simulink model "THSDemo"  (R2023a)
settings: Solver=ode4  StartTime=210  StopTime=260  FixedStep=0.002  RelTol=1e-3
InitFcn:
  |  T_c = 0.002;
undefined symbols (not defined in the file or in its folder): DiscIntNeverNeededParam, Discrete, magnitude, Time
libraries: simulink x23, simulink_extras x8, sharedtransform x3, ctrlSharedLib x2, aerolibconvert2 x1, aerolibtransform2 x1, dspstat3 x1, dspsolvers x1
(part 1 of 2)
settings Model: Creator=zqinghua  LastModifiedBy=LENOVO
settings OptimizationCC: DefaultParameterBehavior=Inlined  OptimizeBlockIOStorage=off  BufferReuse=off  ReuseModelBlockBuffer=off  GlobalBufferReuse=off  ExpressionFolding=off  EnableMemcpy=off  PassReuseOutputArgsAs=Individual arguments  LocalBlockOutputs=off  ZeroExternalMemoryAtStartup=off  ZeroInternalMemoryAtStartup=off  OptimizeDataStoreBuffers=off  BusAssignmentInplaceUpdate=off  OptimizationLevel=level0  OptimizationCustomize=off  EfficientTunableParamExpr=on
settings DebuggingCC: ParameterOverflowMsg=none  ParameterUnderflowMsg=error  ParameterTunabilityLossMsg=error
settings HardwareCC: ProdBitPerInt=16  ProdBitPerPointer=16  ProdBitPerSizeT=16  ProdBitPerPtrDiffT=16  ProdLargestAtomicFloat=None  ProdWordSize=16  ProdHWDeviceType=STMicroelectronics->ST10/Super10  TargetBitPerInt=16  TargetBitPerPointer=16  TargetBitPerSizeT=16  TargetBitPerPtrDiffT=16  TargetIntDivRoundTo=Zero  TargetEndianess=LittleEndian  TargetWordSize=16  TargetHWDeviceType=STMicroelectronics->ST10/Super10
settings SFSimCC: MATLABDynamicMemAlloc=off
settings RTWCC: Description=Embedded Coder  SystemTargetFile=AFCHawk.tlc  GenCodeOnly=on  TemplateMakefile=ert_default_tmf
settings CodeAppCC: ForceParamTrailComments=on  IgnoreCustomStorageClasses=off  OperatorAnnotations=on  SimulinkDataObjDesc=on  SFDataObjDesc=on  InsertBlockDesc=on
settings STFCustomTargetCC: MultiwordLength=256  ModelReferenceCompliant=off  ConcurrentExecutionCompliant=off  CombineOutputUpdateFcns=on  ERTCustomFileBanners=on  SupportContinuousTime=off  SupportNonInlinedSFcns=off  RemoveResetFunc=on  MATLABClassNameForMDSCustomization=Simulink.SoftwareTarget.ERTCustomization  GRTInterface=off  UseToolchainInfoCompliant=off  SystemTargetFile=AFCHawk.tlc
settings ERTTargetCC: TargetLangStandard=C99 (ISO)  ModelReferenceCompliant=off  ParMdlRefBuildCompliant=off  CompOptLevelCompliant=off  ConcurrentExecutionCompliant=off  ModelStepFunctionPrototypeControlCompliant=off  CPPClassGenCompliant=off  UseToolchainInfoCompliant=off  InlinedParameterPlacement=NonHierarchical  ERTCustomFileTemplate=example_file_process.tlc

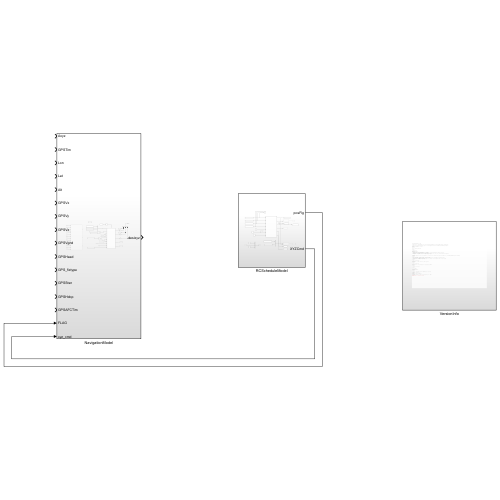
[thumbnail: Simulink's stored preview of the top-level diagram]
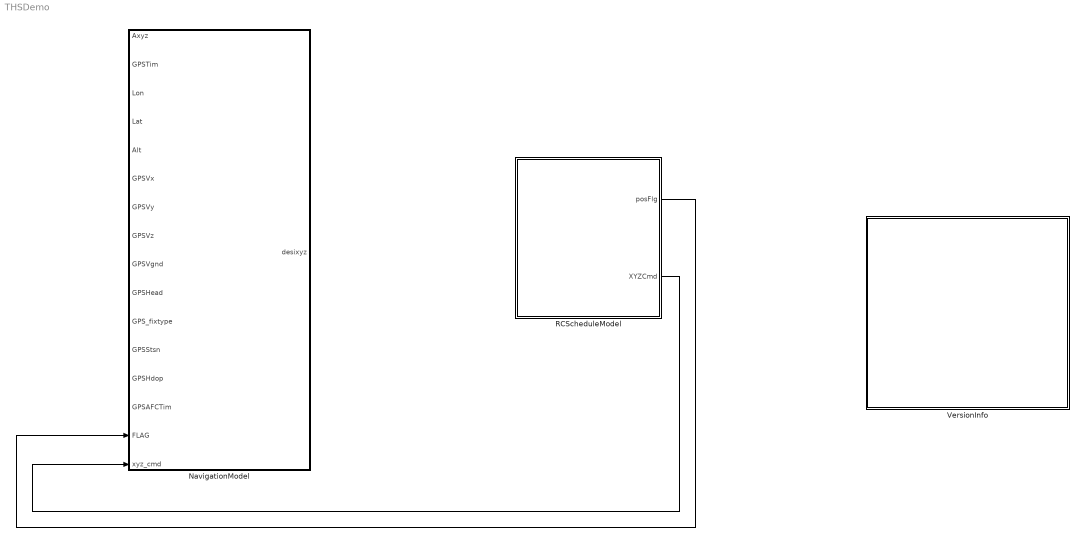
== system THSDemo ==
  NavigationModel : Subsystem
  RCScheduleModel : Subsystem
  VersionInfo : Subsystem
  wires:
  RCScheduleModel/2(XYZCmd) -> NavigationModel/16(xyz_cmd)
  RCScheduleModel/1(posFlg) -> NavigationModel/15(FLAG)

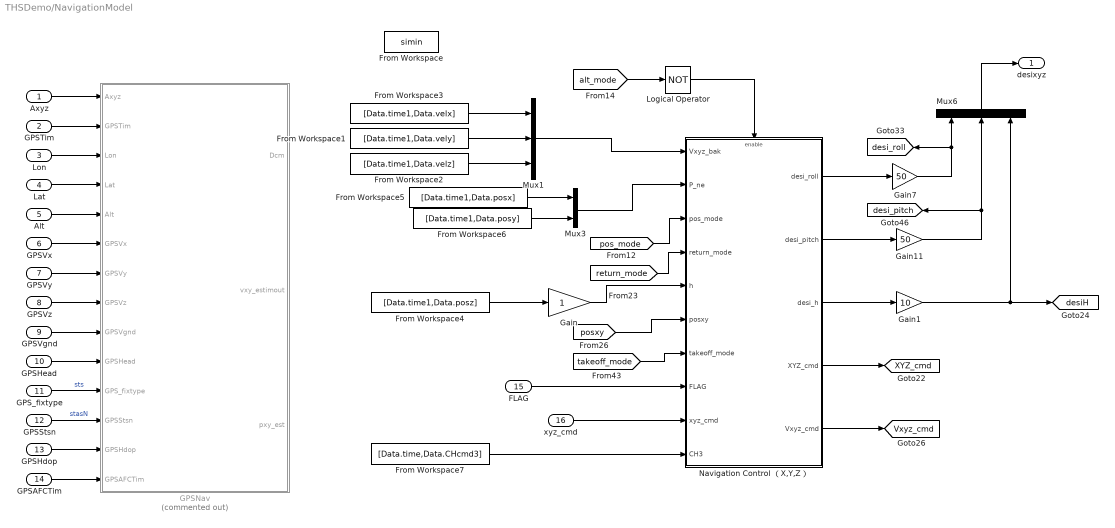
== system THSDemo/NavigationModel ==
  Axyz : Inport
  GPSTim : Inport  Port=2
  Lon : Inport  Port=3
  Lat : Inport  Port=4
  Alt : Inport  Port=5
  GPSVx : Inport  Port=6
  GPSVy : Inport  Port=7
  GPSVz : Inport  Port=8
  GPSVgnd : Inport  Port=9
  GPSHead : Inport  Port=10
  GPS_fixtype : Inport  Port=11
  GPSStsn : Inport  Port=12
  GPSHdop : Inport  Port=13
  GPSAFCTim : Inport  Port=14
  FLAG : Inport  Port=15
  xyz_cmd : Inport  Port=16
  " Navigation Control （X,Y,Z）" : Subsystem
  From Workspace : FromWorkspace  VariableName=simin
  From Workspace1 : FromWorkspace  VariableName=[Data.time1,Data.vely]
  From Workspace2 : FromWorkspace  VariableName=[Data.time1,Data.velz]
  From Workspace3 : FromWorkspace  VariableName=[Data.time1,Data.velx]
  From Workspace4 : FromWorkspace  VariableName=[Data.time1,Data.posz]
  From Workspace5 : FromWorkspace  VariableName=[Data.time1,Data.posx]
  From Workspace6 : FromWorkspace  VariableName=[Data.time1,Data.posy]
  From Workspace7 : FromWorkspace  VariableName=[Data.time,Data.CHcmd3]
  GPSNav : Subsystem  Commented=on
  Gain : Gain
  Gain1 : Gain  Gain=10
  Gain11 : Gain  Gain=50
  Gain7 : Gain  Gain=50
  Logical Operator : Logic  Operator=NOT  AllPortsSameDT=off  OutDataTypeStr=boolean
  Mux1 : Mux  Inputs=3
  Mux3 : Mux  Inputs=2
  Mux6 : Mux  Inputs=3
  desixyz : Outport
  tag scope: Vxyz_cmd=global, XYZ_cmd=global, desiH=global, desi_pitch=global, desi_roll=global
  wires:
  xyz_cmd/1 -> " Navigation Control （X,Y,Z）"/9(xyz_cmd)
  Mux6/1 -> desixyz/1
  FLAG/1 -> " Navigation Control （X,Y,Z）"/8(FLAG)
  Gain1/1 -> Mux6/3, [desiH]
  From Workspace4/1 -> Gain/1
  [takeoff_mode] -> " Navigation Control （X,Y,Z）"/7(takeoff_mode)
  " Navigation Control （X,Y,Z）"/3(desi_h) -> Gain1/1
  [pos_mode] -> " Navigation Control （X,Y,Z）"/3(pos_mode)
  Logical Operator/1 -> " Navigation Control （X,Y,Z）"/Enable
  [return_mode] -> " Navigation Control （X,Y,Z）"/4(return_mode)
  Gain/1 -> " Navigation Control （X,Y,Z）"/5(h)
  [posxy] -> " Navigation Control （X,Y,Z）"/6(posxy)
  " Navigation Control （X,Y,Z）"/1(desi_roll) -> Gain7/1
  " Navigation Control （X,Y,Z）"/2(desi_pitch) -> Gain11/1
  " Navigation Control （X,Y,Z）"/4(XYZ_cmd) -> [XYZ_cmd]
  " Navigation Control （X,Y,Z）"/5(Vxyz_cmd) -> [Vxyz_cmd]
  Gain7/1 -> Mux6/1, [desi_roll]
  Gain11/1 -> Mux6/2, [desi_pitch]
  GPSTim/1 -> GPSNav/2(GPSTim)
  Lon/1 -> GPSNav/3(Lon)
  Lat/1 -> GPSNav/4(Lat)
  Alt/1 -> GPSNav/5(Alt)
  GPSVx/1 -> GPSNav/6(GPSVx)
  GPSVy/1 -> GPSNav/7(GPSVy)
  GPSVz/1 -> GPSNav/8(GPSVz)
  GPSVgnd/1 -> GPSNav/9(GPSVgnd)
  GPSHead/1 -> GPSNav/10(GPSHead)
  GPS_fixtype/1 -> GPSNav/11(GPS_fixtype)  "sts"
  GPSStsn/1 -> GPSNav/12(GPSStsn)  "stasN"
  GPSHdop/1 -> GPSNav/13(GPSHdop)
  GPSAFCTim/1 -> GPSNav/14(GPSAFCTim)
  [alt_mode] -> Logical Operator/1
  Axyz/1 -> GPSNav/1(Axyz)
  From Workspace7/1 -> " Navigation Control （X,Y,Z）"/10(CH3)
  Mux1/1 -> " Navigation Control （X,Y,Z）"/1(Vxyz_bak)
  From Workspace3/1 -> Mux1/1
  From Workspace1/1 -> Mux1/2
  From Workspace2/1 -> Mux1/3
  Mux3/1 -> " Navigation Control （X,Y,Z）"/2(P_ne)
  From Workspace6/1 -> Mux3/2
  From Workspace5/1 -> Mux3/1

== system THSDemo/RCScheduleModel ==
  Constant{,4,7..10} (6 alike) : Constant  Value=0
  From Workspace1 : FromWorkspace  VariableName=[Data.time,Data.ch5]
  From Workspace2 : FromWorkspace  VariableName=[Data.time,Data.ch6]
  From Workspace3 : FromWorkspace  VariableName=[Data.time,Data.ch8]
  From Workspace4 : FromWorkspace  VariableName=[Data.time,Data.ch7]
  From Workspace5 : FromWorkspace  VariableName=[Data.time1,Data.posx]
  From Workspace6 : FromWorkspace  VariableName=[Data.time1,Data.posy]
  Goto27 : Goto  Commented=on  GotoTag=pos_mode_alt
  Goto28 : Goto  Commented=on  GotoTag=posz
  Mux2 : Mux  Inputs=3
  Mux3 : Mux  Inputs=2
  Scope : Scope  NumInputPorts=4
  Subsystem : Subsystem  Commented=on
  Subsystem1 : Subsystem  Commented=on
  control_mode : Subsystem
  posFlg : Outport
  XYZCmd : Outport  Port=2
  tag scope: alt_mode=global, pos_mode=global, posxy=global, return_mode=global, sbus_init_ESC=global, takeoff_mode=global
  wires:
  Mux3/1 -> Subsystem/1(pos)
  Constant/1 -> posFlg/1, control_mode/6(pos_flag)
  Constant7/1 -> Mux2/2
  Constant4/1 -> Mux2/1
  Constant8/1 -> Mux2/3
  From Workspace3/1 -> Scope/4, control_mode/1(sbus_return)
  control_mode/4(pos_mode_alt) -> Goto27/1
  control_mode/3(takeoff_mode) -> [takeoff_mode], Subsystem1/2(pos_mode_0)
  From Workspace4/1 -> Scope/3, control_mode/2(sbus_pos)
  From Workspace2/1 -> Scope/2, control_mode/3(sbus_alt)
  control_mode/1(return_mode) -> Subsystem/2(return), [return_mode]
  control_mode/2(pos_mode) -> [pos_mode]
  control_mode/5(master_alt_mode) -> [alt_mode]
  control_mode/6(sbus_init&ESC1) -> [sbus_init_ESC]
  Subsystem1/1(posz) -> Goto28/1
  Subsystem/1(posxy) -> [posxy]
  Mux2/1 -> XYZCmd/1
  Constant9/1 -> control_mode/5(return_flag)
  Constant10/1 -> control_mode/7(take_off_flag)
  From Workspace5/1 -> Mux3/1
  From Workspace6/1 -> Mux3/2
  From Workspace1/1 -> Scope/1, control_mode/4(sbus_init&ESC)

== system THSDemo/VersionInfo ==
  note: % 2024-01-11 Positon Controller 修改 ， by REZ
      |
      | 1.积分器重置条件，根据油门，已知实际遥控器CH3>0.4左右开始离地，离地前需要进行积分器重置； 遥控器的CH3=0.3-0.4左右对应在模型中Cmd_ch3=880，即重置条件为：当Ch3<880进行积分重置。
      |
      | 2.积分器的限幅范围：对位置控制器里的四个积分器暂时施加了[-3,3]的限幅，主要考虑当x和y方向的位置误差最大在3m内的时候，单纯由积分器得到的控制量不能占据PID控制器主导量而导致控制异常！
      |
      | %2024-01-15:
      | 位置控制器重修，P-PID控制器参数修改了一版；积分限幅
      |
      | % 2024-01-16：
      | 修改增加了一个含逻辑切换的正方形航迹规划指令；
      |
      | %2024-01-19:
      | 航迹规划的优化及飞行验证；
      |
      | %22024-03-08：
      | 增加control_mode模式选择模块：
      | （1）ch5为sbus_init_ESC开关同时进行电调控制解锁与导航初始化，其不受其他模式影响；
      | （2）ch6为高度控制与位置模式的切换通道，通道置1为高度控制模式，否则将进行位置控制模式，在所有模式中高度控制模式优先级最高，只要该通道置1，其他模式将不起作用；
      | （3）ch7为位置控制模式，该模式优先级最低，主要进行航迹飞行，其他通道置零，ch7通道置1，进行预设点飞行，否则进入（0,0,h）定点模式，定点模式可以理解为航迹规划前的无人机位置调整与准备；
      | （4）ch8为返航控制模式，该模式优先级高于航迹控制，但低于高度控制模式，通道置1，无人机将进行返航任务。
      |
      | %22024-03-08：
      | 优化位置控制模块，可随意更改航迹点，并预留与上位机进行点位设置的接口模块。 注意 ，该版本航迹飞行为平面飞行，未涉及到高度，因此在进行点位设置时，只需设计X和Y两个方向的点位，可自行在setpoints封装模块的MASK界面进行修改，同时可修改触发阈值。
      |
      | %22024-03-10：
      | 优化位置控制，同时增加返航模块。将位置控制模式划分为三个模 式，（0,0）定点模式，航迹规划模式，一键返航模式，与control_mode相对应，通过遥控器对应拨杆进行模式切换。
      | （1）三个模式共用同一组控制参数，（0,0）定点模式和航迹规划模式不进行高度控制，保持当前高度；
      | （2）一键返航模式任务要求，无人机接收到指令后，首先保持水平位置，进行高度方向的飞行，达到决断高度之后，无人机保持当前高度h0,然后向（0,0,h）点位飞行，随后无人机进行降落。
      | （3）将位置模式产生的上升率与下降率叠加到遥控器指令生成的控制率中。
      |
      | %22024-03-11：
      | 优化位置控制，可进行三维空间点位设置。
      |
      | %22024-03-12：
      | 取消pos_mode(0,0)模式，优化三维航迹，无人机接受指令后，先飞行高度，随后进行水平飞行。
      |
      | %22024-03-14：
      | 优化返航模式，解决了返航复飞的现象。
      |
      | %22024-03-14：
      | 增加了定点模式，航迹飞行前，无人机先进行当前高度的单定点飞行，验证其飞行性能，随后进行三维航迹飞行。
      |
      | %22024-03-14：
      | 加入偏航控制模式，使其一直处于正北方向。
      |
      | %22024-03-15：
      | 增加上位机点位设置模块。
      |
      | %22024-03-16：
      | 将偏航控制单独加到位置控制模式；
      |
      | %22024-03-17：
      | 增加一键起飞模式，无人机解锁，同时油门至中位，此时，将遥控器7号拨杆至中位，无人机进行一键起飞。
      |
      | %22024-03-18：
      | 简化三维航迹飞行，同时进行高度与水平飞行。
      | %22024-03-22：
      | 优化偏航控制，在飞行高度大于0.5米，偏航控制有效。
      | %22024-03-24：
      | 优化上位机控制逻辑，实现遥控控制与上位机控制相互兼容，上位机可发送起飞指令，返航指令，三维坐标点。
      | %22024-05-15:
      | F550-4 飞8m；未加磁力计补偿，yaw的kp参数需要在线调参为6.6；

== system THSDemo/NavigationModel/ Navigation Control （X,Y,Z） ==
  Vxyz_bak : Inport
  P_ne : Inport  Port=2
  pos_mode : Inport  Port=3
  return_mode : Inport  Port=4
  h : Inport  Port=5
  posxy : Inport  Port=6
  takeoff_mode : Inport  Port=7
  FLAG : Inport  Port=8
  xyz_cmd : Inport  Port=9
  CH3 : Inport  Port=10
  Enable : EnablePort
  POS_CONTROL : Subsystem
  POS_PID : Subsystem
  SETPOINT_z1 : Subsystem
  Scope : Scope  NumInputPorts=2
  Scope1 : Scope  NumInputPorts=2
  desi_roll : Outport
  desi_pitch : Outport  Port=2
  desi_h : Outport  Port=3
  XYZ_cmd : Outport  Port=4
  Vxyz_cmd : Outport  Port=5
  wires:
  POS_PID/1(desi_roll) -> desi_roll/1
  POS_PID/2(desi_pitch) -> desi_pitch/1
  POS_PID/3(desi_h) -> desi_h/1
  return_mode/1 -> SETPOINT_z1/3(return_mode)
  pos_mode/1 -> SETPOINT_z1/2(pos_mode)
  SETPOINT_z1/1(XYZ_cmd) -> POS_CONTROL/1(XYZ_cmd), Scope1/1, XYZ_cmd/1
  P_ne/1 -> SETPOINT_z1/4(pos), Scope1/2, POS_CONTROL/2(pos)
  h/1 -> POS_CONTROL/3(h), SETPOINT_z1/5(h)
  POS_CONTROL/1(Vxyz_cmd) -> POS_PID/1(Vxyz_cmd), Scope/1, Vxyz_cmd/1
  posxy/1 -> SETPOINT_z1/1(posxy)
  takeoff_mode/1 -> SETPOINT_z1/6(takeoff_mode)
  xyz_cmd/1 -> SETPOINT_z1/7(xyz_cmd)
  FLAG/1 -> SETPOINT_z1/8(FLAG)
  CH3/1 -> POS_PID/3(CH3)
  Vxyz_bak/1 -> Scope/2, POS_PID/2(Vxyz_bak)

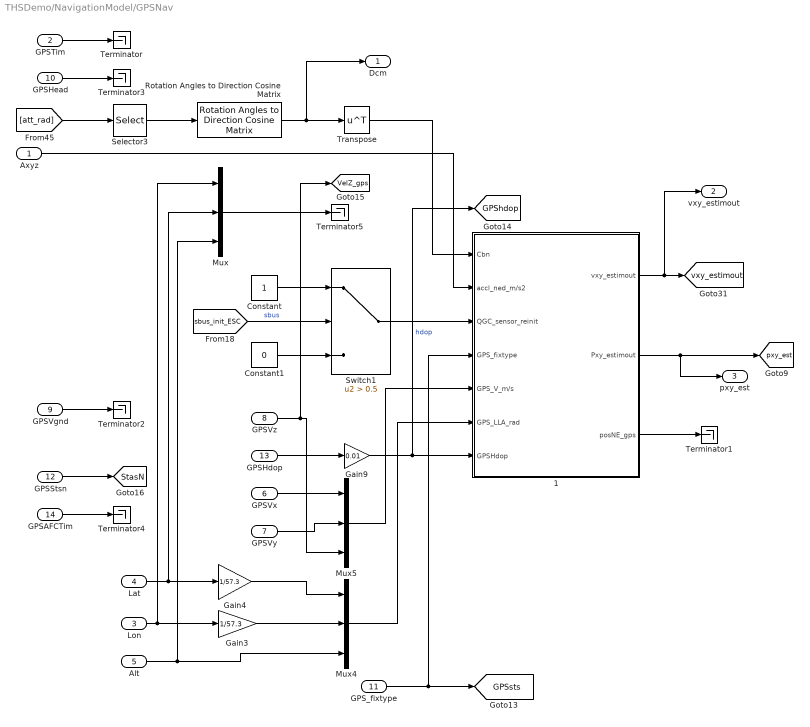
== system THSDemo/NavigationModel/GPSNav ==
  Axyz : Inport
  GPSTim : Inport  Port=2
  Lon : Inport  Port=3
  Lat : Inport  Port=4
  Alt : Inport  Port=5
  GPSVx : Inport  Port=6
  GPSVy : Inport  Port=7
  GPSVz : Inport  Port=8
  GPSVgnd : Inport  Port=9
  GPSHead : Inport  Port=10
  GPS_fixtype : Inport  Port=11
  GPSStsn : Inport  Port=12
  GPSHdop : Inport  Port=13
  GPSAFCTim : Inport  Port=14
  1 : Subsystem  mask{dt=0.002}
      mask prompts: dt "步长"
      mask DialogControl ParameterGroupVar Prompt: 参数
  Constant : Constant
  Constant1 : Constant  Value=0
  Gain3 : Gain  Gain=1/57.3
  Gain4 : Gain  Gain=1/57.3
  Gain9 : Gain  Gain=0.01
  Mux : Mux  Inputs=3
  Mux4 : Mux  Inputs=3
  Mux5 : Mux  Inputs=3
  Rotation Angles to Direction Cosine Matrix : sharedtransform/Rotation Angles to Direction Cosine Matrix  rotationOrder=ZYX  aMode=aMode
  Selector3 : Selector  InputPortWidth=3  IndexOptions=Index vector (dialog)  Indices=[3 2 1]  OutputSizes=1
  Switch1 : Switch  Criteria=u2 > Threshold  Threshold=0.5  SaturateOnIntegerOverflow=off  InputSameDT=off
  Terminator{,1..5} (6 alike) : Terminator
  Transpose : Math  Operator=transpose
  Dcm : Outport
  vxy_estimout : Outport  Port=2
  pxy_est : Outport  Port=3
  tag scope: GPShdop=global, GPSsts=global, StasN=global, VelZ_gps=global, pxy_est=global, vxy_estimout=global
  wires:
  GPSTim/1 -> Terminator/1
  GPSVz/1 -> [VelZ_gps], Mux5/3
  GPSStsn/1 -> [StasN]
  GPSVgnd/1 -> Terminator2/1
  GPSHead/1 -> Terminator3/1
  Gain3/1 -> Mux4/2
  Mux/1 -> Terminator5/1
  [att_rad] -> Selector3/1
  Selector3/1 -> Rotation Angles to Direction Cosine Matrix/1
  Axyz/1 -> 1/2(accl_ned_m/s2)
  GPSAFCTim/1 -> Terminator4/1
  Lat/1 -> Gain4/1, Mux/2
  GPSVy/1 -> Mux5/2
  Lon/1 -> Gain3/1, Mux/1
  Alt/1 -> Mux4/3, Mux/3
  Rotation Angles to Direction Cosine Matrix/1 -> Transpose/1, Dcm/1
  Constant1/1 -> Switch1/3
  [sbus_init_ESC] -> Switch1/2  "sbus"
  Constant/1 -> Switch1/1
  GPSHdop/1 -> Gain9/1
  GPSVx/1 -> Mux5/1
  Gain4/1 -> Mux4/1
  Transpose/1 -> 1/1(Cbn)
  Switch1/1 -> 1/3(QGC_sensor_reinit)
  Mux4/1 -> 1/6(GPS_LLA_rad)
  Gain9/1 -> 1/7(GPSHdop), [GPShdop]  "hdop"
  Mux5/1 -> 1/5(GPS_V_m/s)
  GPS_fixtype/1 -> [GPSsts], 1/4(GPS_fixtype)
  1/1(vxy_estimout) -> [vxy_estimout], vxy_estimout/1
  1/2(Pxy_estimout) -> pxy_est/1, [pxy_est]
  1/3(posNE_gps) -> Terminator1/1

== system THSDemo/RCScheduleModel/Subsystem ==
  pos : Inport
  return : Inport  Port=2
  Logical Operator : Logic  Operator=NOT  AllPortsSameDT=off  OutDataTypeStr=boolean
  Memory : Memory
  Switch : Switch  Criteria=u2 > Threshold  Threshold=0.5  SaturateOnIntegerOverflow=off  InputSameDT=off
  posxy : Outport
  wires:
  Switch/1 -> Memory/1, posxy/1
  Memory/1 -> Switch/3
  return/1 -> Logical Operator/1
  pos/1 -> Switch/1
  Logical Operator/1 -> Switch/2

== system THSDemo/RCScheduleModel/Subsystem1 ==
  h : Inport
  pos_mode_0 : Inport  Port=2
  Gain : Gain  Gain=-0.01
  Logical Operator : Logic  Operator=NOT  AllPortsSameDT=off  OutDataTypeStr=boolean
  Memory : Memory
  Switch : Switch  Criteria=u2 > Threshold  Threshold=0.5  SaturateOnIntegerOverflow=off  InputSameDT=off
  posz : Outport
  wires:
  Logical Operator/1 -> Switch/2
  h/1 -> Gain/1
  pos_mode_0/1 -> Logical Operator/1
  Memory/1 -> Switch/3
  Switch/1 -> posz/1, Memory/1
  Gain/1 -> Switch/1

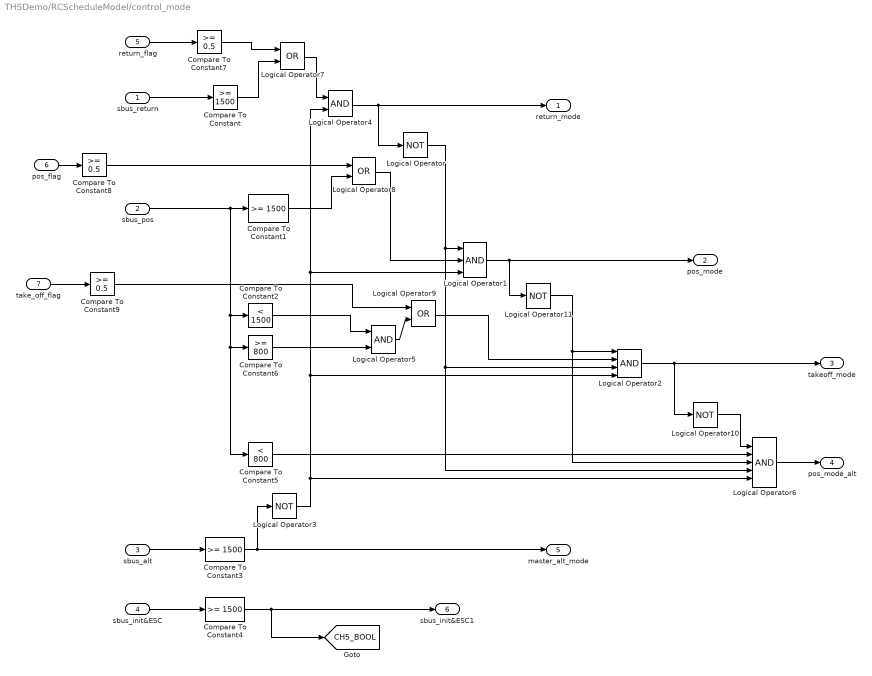
== system THSDemo/RCScheduleModel/control_mode ==
  sbus_return : Inport
  sbus_pos : Inport  Port=2
  sbus_alt : Inport  Port=3
  sbus_init&ESC : Inport  Port=4
  return_flag : Inport  Port=5
  pos_flag : Inport  Port=6
  take_off_flag : Inport  Port=7
  Compare To Constant{,1,3..4} (4 alike) : simulink/Logic and Bit Operations/Compare To Constant  relop=>=  const=1500  OutDataTypeStr=boolean
  Compare To Constant2 : simulink/Logic and Bit Operations/Compare To Constant  relop=<  const=1500  OutDataTypeStr=boolean
  Compare To Constant5 : simulink/Logic and Bit Operations/Compare To Constant  relop=<  const=800  OutDataTypeStr=boolean
  Compare To Constant6 : simulink/Logic and Bit Operations/Compare To Constant  relop=>=  const=800  OutDataTypeStr=boolean
  Compare To Constant7 : simulink/Logic and Bit Operations/Compare To Constant  relop=>=  const=0.5  OutDataTypeStr=boolean
  Compare To Constant8 : simulink/Logic and Bit Operations/Compare To Constant  relop=>=  const=0.5  OutDataTypeStr=boolean
  Compare To Constant9 : simulink/Logic and Bit Operations/Compare To Constant  relop=>=  const=0.5  OutDataTypeStr=boolean
  Logical Operator{,3,10..11} (4 alike) : Logic  Operator=NOT  AllPortsSameDT=off  OutDataTypeStr=boolean
  Logical Operator1 : Logic  Inputs=3  AllPortsSameDT=off  OutDataTypeStr=boolean
  Logical Operator2 : Logic  Inputs=4  AllPortsSameDT=off  OutDataTypeStr=boolean
  Logical Operator4 : Logic  AllPortsSameDT=off  OutDataTypeStr=boolean
  Logical Operator5 : Logic  AllPortsSameDT=off  OutDataTypeStr=boolean
  Logical Operator6 : Logic  Inputs=5  AllPortsSameDT=off  OutDataTypeStr=boolean
  Logical Operator7 : Logic  Operator=OR  AllPortsSameDT=off  OutDataTypeStr=boolean
  Logical Operator8 : Logic  Operator=OR  AllPortsSameDT=off  OutDataTypeStr=boolean
  Logical Operator9 : Logic  Operator=OR  AllPortsSameDT=off  OutDataTypeStr=boolean
  return_mode : Outport
  pos_mode : Outport  Port=2
  takeoff_mode : Outport  Port=3
  pos_mode_alt : Outport  Port=4
  master_alt_mode : Outport  Port=5
  sbus_init&ESC1 : Outport  Port=6
  tag scope: CH5_BOOL=global
  wires:
  Logical Operator4/1 -> Logical Operator/1, return_mode/1
  Logical Operator/1 -> Logical Operator6/4, Logical Operator2/3, Logical Operator1/1
  sbus_return/1 -> Compare To Constant/1
  Compare To Constant1/1 -> Logical Operator8/2
  Logical Operator1/1 -> pos_mode/1, Logical Operator11/1
  Compare To Constant2/1 -> Logical Operator5/1
  Logical Operator2/1 -> Logical Operator10/1, takeoff_mode/1
  sbus_alt/1 -> Compare To Constant3/1
  Compare To Constant3/1 -> master_alt_mode/1, Logical Operator3/1
  Compare To Constant/1 -> Logical Operator7/2
  Logical Operator3/1 -> Logical Operator4/2, Logical Operator1/3, Logical Operator2/4, Logical Operator6/5
  sbus_init&ESC/1 -> Compare To Constant4/1
  Compare To Constant4/1 -> [CH5_BOOL], sbus_init&ESC1/1
  Compare To Constant5/1 -> Logical Operator6/2
  sbus_pos/1 -> Compare To Constant5/1, Compare To Constant6/1, Compare To Constant2/1, Compare To Constant1/1
  Compare To Constant6/1 -> Logical Operator5/2
  Logical Operator5/1 -> Logical Operator9/2
  Logical Operator6/1 -> pos_mode_alt/1
  return_flag/1 -> Compare To Constant7/1
  Compare To Constant7/1 -> Logical Operator7/1
  Logical Operator7/1 -> Logical Operator4/1
  pos_flag/1 -> Compare To Constant8/1
  Compare To Constant8/1 -> Logical Operator8/1
  Logical Operator8/1 -> Logical Operator1/2
  take_off_flag/1 -> Compare To Constant9/1
  Logical Operator9/1 -> Logical Operator2/2
  Compare To Constant9/1 -> Logical Operator9/1
  Logical Operator10/1 -> Logical Operator6/1
  Logical Operator11/1 -> Logical Operator6/3, Logical Operator2/1

== system THSDemo/NavigationModel/ Navigation Control （X,Y,Z）/POS_CONTROL ==
  note: 位置P控制
  XYZ_cmd : Inport
  pos : Inport  Port=2
  h : Inport  Port=3
  Add1 : Sum  Inputs=+-
  Demux : Demux  Outputs=3
  Gain : Gain
  Mux : Mux  Inputs=3
  Mux1 : Mux  Inputs=2
  POS_P : Gain  Gain=[0.7 0.7 0.8]
  Reshape : Reshape
  Saturation2 : Saturate  UpperLimit=3  LowerLimit=-3
  Saturation3 : Saturate  UpperLimit=3  LowerLimit=-3
  Saturation4 : Saturate  UpperLimit=3  LowerLimit=-3
  Vxyz_cmd : Outport
  wires:
  h/1 -> Gain/1  "h"
  Add1/1 -> Reshape/1
  Gain/1 -> Mux1/2
  pos/1 -> Mux1/1  "XY"
  Mux1/1 -> Add1/2
  XYZ_cmd/1 -> Add1/1  "XYZ_cmd"
  POS_P/1 -> Demux/1
  Mux/1 -> Vxyz_cmd/1
  Demux/1 -> Saturation2/1
  Demux/2 -> Saturation3/1
  Demux/3 -> Saturation4/1
  Saturation2/1 -> Mux/1
  Saturation3/1 -> Mux/2
  Saturation4/1 -> Mux/3
  Reshape/1 -> POS_P/1

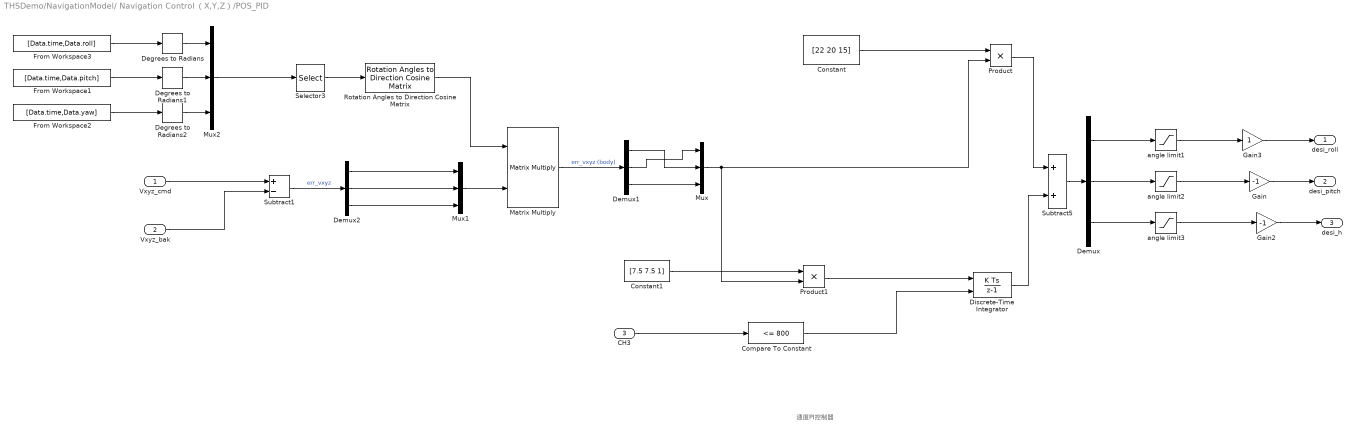
== system THSDemo/NavigationModel/ Navigation Control （X,Y,Z）/POS_PID ==
  note: 速度PI控制器
  Vxyz_cmd : Inport
  Vxyz_bak : Inport  Port=2
  CH3 : Inport  Port=3
  Compare To Constant : simulink/Logic and Bit Operations/Compare To Constant  relop=<=  const=800  OutDataTypeStr=boolean
  Constant : Constant  Value=[22 20 15]
  Constant1 : Constant  Value=[7.5 7.5 1]
  Degrees to Radians : simulink_extras/Transformations/Degrees to Radians
  Degrees to Radians1 : simulink_extras/Transformations/Degrees to Radians
  Degrees to Radians2 : simulink_extras/Transformations/Degrees to Radians
  Demux : Demux  Outputs=3
  Demux1 : Demux  Outputs=3
  Demux2 : Demux  Outputs=3
  Discrete-Time Integrator : DiscreteIntegrator  ExternalReset=level  SampleTime=-1  LimitOutput=on  UpperSaturationLimit=5  LowerSaturationLimit=-5  ICPrevOutput=DiscIntNeverNeededParam  ICPrevScaledInput=DiscIntNeverNeededParam
  From Workspace1 : FromWorkspace  VariableName=[Data.time,Data.pitch]
  From Workspace2 : FromWorkspace  VariableName=[Data.time,Data.yaw]
  From Workspace3 : FromWorkspace  VariableName=[Data.time,Data.roll]
  Gain : Gain  Gain=-1
  Gain2 : Gain  Gain=-1
  Gain3 : Gain
  Matrix Multiply : Product  Multiplication=Matrix(*)
  Mux : Mux  Inputs=3
  Mux1 : Mux  Inputs=3
  Mux2 : Mux  Inputs=3
  Product : Product
  Product1 : Product
  Rotation Angles to Direction Cosine Matrix : sharedtransform/Rotation Angles to Direction Cosine Matrix  rotationOrder=ZYX  aMode=aMode
  Selector3 : Selector  InputPortWidth=3  IndexOptions=Index vector (dialog)  Indices=[3 2 1]  OutputSizes=1
  Subtract1 : Sum  Inputs=+-
  Subtract5 : Sum
  angle limit1 : Saturate  UpperLimit=30  LowerLimit=-30
  angle limit2 : Saturate  UpperLimit=30  LowerLimit=-30
  angle limit3 : Saturate  UpperLimit=20  LowerLimit=-20
  desi_roll : Outport
  desi_pitch : Outport  Port=2
  desi_h : Outport  Port=3
  wires:
  angle limit2/1 -> Gain/1
  Constant1/1 -> Product1/1
  angle limit1/1 -> Gain3/1
  Discrete-Time Integrator/1 -> Subtract5/2
  Demux/1 -> angle limit1/1
  Demux/2 -> angle limit2/1
  Gain/1 -> desi_pitch/1
  Gain3/1 -> desi_roll/1
  Compare To Constant/1 -> Discrete-Time Integrator/2
  Subtract5/1 -> Demux/1
  Gain2/1 -> desi_h/1
  Demux/3 -> angle limit3/1
  angle limit3/1 -> Gain2/1
  Demux1/1 -> Mux/2
  Demux1/2 -> Mux/1
  Demux1/3 -> Mux/3
  Matrix Multiply/1 -> Demux1/1  "err_vxyz (body)"
  Rotation Angles to Direction Cosine Matrix/1 -> Matrix Multiply/1
  Vxyz_cmd/1 -> Subtract1/1
  Vxyz_bak/1 -> Subtract1/2
  Subtract1/1 -> Demux2/1  "err_vxyz"
  Demux2/2 -> Mux1/2
  Demux2/1 -> Mux1/1
  Mux1/1 -> Matrix Multiply/2
  Demux2/3 -> Mux1/3
  Constant/1 -> Product/1
  Mux/1 -> Product1/2, Product/2
  Product/1 -> Subtract5/1
  Product1/1 -> Discrete-Time Integrator/1
  CH3/1 -> Compare To Constant/1
  Selector3/1 -> Rotation Angles to Direction Cosine Matrix/1
  Mux2/1 -> Selector3/1
  Degrees to Radians/1 -> Mux2/1
  Degrees to Radians1/1 -> Mux2/2
  Degrees to Radians2/1 -> Mux2/3
  From Workspace3/1 -> Degrees to Radians/1
  From Workspace1/1 -> Degrees to Radians1/1
  From Workspace2/1 -> Degrees to Radians2/1

== system THSDemo/NavigationModel/ Navigation Control （X,Y,Z）/SETPOINT_z1 ==
  posxy : Inport
  pos_mode : Inport  Port=2
  return_mode : Inport  Port=3
  pos : Inport  Port=4
  h : Inport  Port=5
  takeoff_mode : Inport  Port=6
  xyz_cmd : Inport  Port=7
  FLAG : Inport  Port=8
  Merge : Merge  Inputs=3
  Merge1 : Merge  Inputs=3
  Mux : Mux  Inputs=2
  Scope : Scope
  Subsystem : Subsystem
  return_mode1 : Subsystem  mask{landing_pos=[0 0 0], decision_h=8, accept_radius=0.7, accept_radius_h=0.5}
      mask DialogControl ParameterGroupVar Prompt: 参数
  return_mode2 : Subsystem  Commented=on  mask{landing_pos=[0 0 0], decision_h=8, accept_radius=0.5, accept_radius_h=0.4}
      mask DialogControl ParameterGroupVar Prompt: 参数
  setpoints1 : Subsystem  mask{setpoints=[10 0 -5;10 10 -5;0 10 -5;0 0 -5], accept_radius_1=0.7}
      mask DialogControl ParameterGroupVar Prompt: 参数
  setpoints2 : Subsystem  Commented=on  mask{setpoints=[10 0 -5;10 10 -5;0 10 -5;0 0 -5], accept_radius_1=0.5}
      mask DialogControl ParameterGroupVar Prompt: 参数
  takeoff1 : Subsystem  Commented=on  mask{setpoint1=[0 0], takeoff_h=-5}
      mask DialogControl ParameterGroupVar Prompt: 参数
  takeoff2 : Subsystem  mask{setpoint1=[0 0], takeoff_h=-5}
      mask DialogControl ParameterGroupVar Prompt: 参数
  XYZ_cmd : Outport
  wires:
  posxy/1 -> return_mode1/2(posxy)
  return_mode1/1(setpoint_next) -> Merge/3  "XYZ_cmd"
  Mux/1 -> return_mode1/1(pos1), setpoints1/1(pos1)  "XYZ"
  setpoints1/1(setpoint_next) -> Merge/2  "XYZ_cmd"
  Merge/1 -> XYZ_cmd/1
  return_mode/1 -> return_mode1/Enable
  pos_mode/1 -> setpoints1/Enable
  pos/1 -> Subsystem/2(pos), Mux/1  "XY"
  h/1 -> takeoff2/2(h), Mux/2
  takeoff_mode/1 -> takeoff2/Enable, Subsystem/1(takeoff)
  takeoff2/1(setpoint_next) -> Merge/1  "XYZ_cmd"
  xyz_cmd/1 -> setpoints1/2(xyz_cmd)
  FLAG/1 -> setpoints1/3(FLAG)
  Subsystem/1(posxy) -> takeoff2/1(posxy)
  takeoff2/2(flag) -> Merge1/1
  setpoints1/2(flag) -> Merge1/2
  return_mode1/2(flag) -> Merge1/3
  Merge1/1 -> Scope/1

== system THSDemo/NavigationModel/GPSNav/1 ==
  Cbn : Inport
  accl_ned_m/s2 : Inport  Port=2
  QGC_sensor_reinit : Inport  Port=3
  GPS_fixtype : Inport  Port=4
  GPS_V_m/s : Inport  Port=5
  GPS_LLA_rad : Inport  Port=6
  GPSHdop : Inport  Port=7
  Cast To Boolean : DataTypeConversion  OutDataTypeStr=double  SaturateOnIntegerOverflow=off  RndMeth=Floor
  Compare To Constant : simulink/Logic and Bit Operations/Compare To Constant  relop=>=  const=1  OutDataTypeStr=boolean
  Compare To Constant1 : simulink/Logic and Bit Operations/Compare To Constant  relop=>=  const=1  OutDataTypeStr=boolean
  GPS_Data_Process : Subsystem
  Logical Operator : Logic  AllPortsSameDT=off  OutDataTypeStr=boolean
  Translation_estimate : Subsystem
  vxy_estimout : Outport
  Pxy_estimout : Outport  Port=2
  posNE_gps : Outport  Port=3
  tag scope: AccelFusion_sta=global
  wires:
  Compare To Constant/1 -> Logical Operator/1
  GPS_Data_Process/1(init_GPSLLAflag) -> Compare To Constant1/1
  GPSHdop/1 -> Translation_estimate/6(GPSHdop), GPS_Data_Process/5(GPSHdop)
  QGC_sensor_reinit/1 -> Translation_estimate/7(QGC_init), GPS_Data_Process/4(QGC_sensor_reinit)
  GPS_LLA_rad/1 -> GPS_Data_Process/2(GPS_LLA_rad)
  GPS_V_m/s/1 -> GPS_Data_Process/1(GPS_V_m/s)
  accl_ned_m/s2/1 -> Translation_estimate/2(accl_ned_m/s2)
  Cbn/1 -> Translation_estimate/1(Cbn)
  GPS_Data_Process/2(vne_gps) -> Translation_estimate/3(vne_gps)
  GPS_Data_Process/3(posNE_gps) -> posNE_gps/1, Translation_estimate/4(posNE_gps1)
  GPS_fixtype/1 -> Compare To Constant/1, Translation_estimate/5(GPSstate), GPS_Data_Process/3(GPS_fixtype)  "sts"
  Translation_estimate/1(vxy_estimout) -> vxy_estimout/1
  Translation_estimate/2(Pxy_estimout) -> Pxy_estimout/1
  Cast To Boolean/1 -> [AccelFusion_sta]
  Compare To Constant1/1 -> Logical Operator/2
  Logical Operator/1 -> Translation_estimate/Enable, Cast To Boolean/1

== system THSDemo/NavigationModel/ Navigation Control （X,Y,Z）/SETPOINT_z1/Subsystem ==
  takeoff : Inport
  pos : Inport  Port=2
  Logical Operator : Logic  Operator=NOT  AllPortsSameDT=off  OutDataTypeStr=boolean
  Memory : Memory
  Switch : Switch  Criteria=u2 > Threshold  Threshold=0.5  SaturateOnIntegerOverflow=off  InputSameDT=off
  posxy : Outport
  wires:
  Switch/1 -> Memory/1, posxy/1
  Memory/1 -> Switch/3
  takeoff/1 -> Logical Operator/1
  pos/1 -> Switch/1
  Logical Operator/1 -> Switch/2

== system THSDemo/NavigationModel/ Navigation Control （X,Y,Z）/SETPOINT_z1/return_mode1 ==
  pos1 : Inport
  posxy : Inport  Port=2  PortDimensions=[ 2 1]
  Enable : EnablePort
  Abs : Abs  SaturateOnIntegerOverflow=off
  Add1 : Sum  Inputs=+-
  Add4 : Sum  Inputs=+-
  Constant : Constant  Value=landing_pos
  Constant1 : Constant  Value=-decision_h
  Constant11 : Constant  Value=10
  Constant2 : Constant  Value=-decision_h
  Constant3 : Constant  Value=accept_radius_h
  Constant4 : Constant  Value=accept_radius
  Logical Operator : Logic  Operator=NOT  AllPortsSameDT=off  OutDataTypeStr=boolean
  Memory{1..4} (4 alike) : Memory
  Mux : Mux  Inputs=2
  Mux1 : Mux  Inputs=2
  Relational Operator1 : RelationalOperator  Operator=<=  OutDataTypeStr=boolean  RndMeth=Simplest  InputSameDT=off
  Relational Operator2 : RelationalOperator  Operator=<=  OutDataTypeStr=boolean  RndMeth=Simplest  InputSameDT=off
  Selector1 : Selector  InputPortWidth=3  IndexOptions=Index vector (dialog)  Indices=[3]  OutputSizes=1
  Selector6 : Selector  InputPortWidth=3  IndexOptions=Index vector (dialog)  Indices=[1 2]  OutputSizes=1
  Selector7 : Selector  InputPortWidth=3  IndexOptions=Index vector (dialog)  Indices=[1 2]  OutputSizes=1
  Switch{,1..2,4} (4 alike) : Switch  Criteria=u2 > Threshold  Threshold=0.5  SaturateOnIntegerOverflow=off  InputSameDT=off
  TD : Subsystem
  norm : Subsystem
  setpoint_next : Outport
  flag : Outport  Port=2
  wires:
  TD/1(setpoint_next) -> setpoint_next/1
  Add4/1 -> norm/1(u)
  Mux1/1 -> Switch1/1
  norm/1(y) -> Switch2/3
  Relational Operator1/1 -> Switch1/2, Memory1/1, Logical Operator/1
  Constant3/1 -> Relational Operator1/2
  posxy/1 -> Mux/1
  Relational Operator2/1 -> Memory3/1, Switch/2
  Selector6/1 -> Add4/1
  Constant2/1 -> Add1/2, Mux/2
  Constant4/1 -> Relational Operator2/2
  Memory1/1 -> Switch4/2
  Selector7/1 -> Add4/2, Mux1/1
  Memory3/1 -> Switch2/2
  Memory4/1 -> Switch2/1
  Mux/1 -> Switch1/3
  Switch2/1 -> Relational Operator2/1, Memory4/1
  Switch1/1 -> Switch/3
  Constant/1 -> Switch/1, Selector7/1
  Constant1/1 -> Mux1/2
  Memory2/1 -> Switch4/1
  Selector1/1 -> Add1/1
  Switch4/1 -> Relational Operator1/1, Memory2/1
  Add1/1 -> Abs/1
  Abs/1 -> Switch4/3
  Switch/1 -> TD/1(D)
  Constant11/1 -> TD/2(r)
  pos1/1 -> TD/3(r1), Selector1/1, Selector6/1
  Logical Operator/1 -> flag/1

== system THSDemo/NavigationModel/ Navigation Control （X,Y,Z）/SETPOINT_z1/return_mode2 ==
  pos1 : Inport
  posxy : Inport  Port=2
  Enable : EnablePort
  Abs : Abs  SaturateOnIntegerOverflow=off
  Add1 : Sum  Inputs=+-
  Add4 : Sum  Inputs=+-
  Constant : Constant  Value=landing_pos
  Constant1 : Constant  Value=-decision_h
  Constant11 : Constant  Value=10
  Constant2 : Constant  Value=-decision_h
  Constant3 : Constant  Value=accept_radius_h
  Constant4 : Constant  Value=accept_radius
  Memory{1..4} (4 alike) : Memory
  Mux : Mux  Inputs=2
  Mux1 : Mux  Inputs=2
  Relational Operator1 : RelationalOperator  Operator=<=  OutDataTypeStr=boolean  RndMeth=Simplest  InputSameDT=off
  Relational Operator2 : RelationalOperator  Operator=<=  OutDataTypeStr=boolean  RndMeth=Simplest  InputSameDT=off
  Selector1 : Selector  InputPortWidth=3  IndexOptions=Index vector (dialog)  Indices=[3]  OutputSizes=1
  Selector6 : Selector  InputPortWidth=3  IndexOptions=Index vector (dialog)  Indices=[1 2]  OutputSizes=1
  Selector7 : Selector  InputPortWidth=3  IndexOptions=Index vector (dialog)  Indices=[1 2]  OutputSizes=1
  Signal Conversion : SignalConversion  OverrideOpt=off
  Switch{,1..2,4} (4 alike) : Switch  Criteria=u2 > Threshold  Threshold=0.5  SaturateOnIntegerOverflow=off  InputSameDT=off
  TD : Subsystem
  norm : Subsystem
  setpoint_next : Outport
  wires:
  pos1/1 -> Selector6/1, Selector1/1, TD/3(r1)
  Constant11/1 -> TD/2(r)
  Switch/1 -> Signal Conversion/1
  Signal Conversion/1 -> TD/1(D)
  Abs/1 -> Switch4/3
  Add1/1 -> Abs/1
  Switch4/1 -> Memory2/1, Relational Operator1/1
  Selector1/1 -> Add1/1
  Memory2/1 -> Switch4/1
  Constant1/1 -> Mux1/2
  Constant/1 -> Selector7/1, Switch/1
  Switch1/1 -> Switch/3
  Switch2/1 -> Memory4/1, Relational Operator2/1
  Mux/1 -> Switch1/3
  Memory4/1 -> Switch2/1
  Memory3/1 -> Switch2/2
  Selector7/1 -> Mux1/1, Add4/2
  Memory1/1 -> Switch4/2
  Constant4/1 -> Relational Operator2/2
  Constant2/1 -> Mux/2, Add1/2
  Selector6/1 -> Add4/1
  Relational Operator2/1 -> Switch/2, Memory3/1
  posxy/1 -> Mux/1
  Constant3/1 -> Relational Operator1/2
  Relational Operator1/1 -> Memory1/1, Switch1/2
  norm/1(y) -> Switch2/3
  Mux1/1 -> Switch1/1
  Add4/1 -> norm/1(u)
  TD/1(setpoint_next) -> setpoint_next/1

== system THSDemo/NavigationModel/ Navigation Control （X,Y,Z）/SETPOINT_z1/setpoints1 ==
  pos1 : Inport
  xyz_cmd : Inport  Port=2
  FLAG : Inport  Port=3
  Enable : EnablePort
  Add : Sum
  Add2 : Sum
  Chart : Stateflow chart  TreatAsAtomicUnit=on
  Constant1 : Constant
  Constant11 : Constant  Value=10
  Constant2 : Constant  Value=0
  Constant3 : Constant
  Constant4 : Constant  Value=accept_radius_1
  Constant5 : Constant  Value=setpoints
  Logical Operator : Logic  Operator=OR  AllPortsSameDT=off  OutDataTypeStr=boolean
  Memory : Memory  InheritSampleTime=on
  Relational Operator2 : RelationalOperator  Operator=<=  OutDataTypeStr=boolean  RndMeth=Simplest  InputSameDT=off
  Saturation : Saturate  UpperLimit=size(setpoints,1)  LowerLimit=1
  Selector1 : Selector  NumberOfDimensions=2  InputPortWidth=4  IndexOptions=Index vector (port),Select all  Indices=[1 3],1  OutputSizes=1,1
  Subtract : Sum  Inputs=+-
  Switch : Switch  Criteria=u2 > Threshold  SaturateOnIntegerOverflow=off  InputSameDT=off
  Switch5 : Switch  Criteria=u2 > Threshold  Threshold=0.5  SaturateOnIntegerOverflow=off  InputSameDT=off
  TD : Subsystem
  Transpose1 : Math  Operator=transpose  SignedPower=on
  norm : Subsystem
  setpoint_next : Outport
  flag : Outport  Port=2
  wires:
  Relational Operator2/1 -> Chart/1(dist)
  norm/1(y) -> Relational Operator2/1
  Selector1/1 -> Transpose1/1
  Constant3/1 -> Add2/2
  Add/1 -> Memory/1
  Saturation/1 -> Selector1/2
  Constant4/1 -> Relational Operator2/2
  Constant1/1 -> Switch/1
  Memory/1 -> Add/2, Add2/1
  Constant2/1 -> Switch/3
  Switch/1 -> Add/1
  Add2/1 -> Saturation/1
  Subtract/1 -> norm/1(u)
  Chart/1(flag_setpoint) -> Logical Operator/1, Switch/2
  Constant5/1 -> Selector1/1
  xyz_cmd/1 -> Switch5/1
  FLAG/1 -> Logical Operator/2, Switch5/2
  TD/1(setpoint_next) -> setpoint_next/1
  Transpose1/1 -> Subtract/2, Switch5/3
  pos1/1 -> Subtract/1, TD/3(r1)
  Constant11/1 -> TD/2(r)
  Switch5/1 -> TD/1(D)
  Logical Operator/1 -> flag/1

== system THSDemo/NavigationModel/ Navigation Control （X,Y,Z）/SETPOINT_z1/setpoints2 ==
  pos1 : Inport
  xyz_cmd : Inport  Port=2
  FLAG : Inport  Port=3
  Enable : EnablePort
  Add : Sum
  Add2 : Sum
  Chart : Stateflow chart  TreatAsAtomicUnit=on
  Constant1 : Constant
  Constant11 : Constant  Value=10
  Constant2 : Constant  Value=0
  Constant3 : Constant
  Constant4 : Constant  Value=accept_radius_1
  Constant5 : Constant  Value=setpoints
  Memory : Memory  InheritSampleTime=on
  Relational Operator2 : RelationalOperator  Operator=<=  OutDataTypeStr=boolean  RndMeth=Simplest  InputSameDT=off
  Saturation : Saturate  UpperLimit=size(setpoints,1)  LowerLimit=1
  Selector1 : Selector  NumberOfDimensions=2  InputPortWidth=4  IndexOptions=Index vector (port),Select all  Indices=[1 3],1  OutputSizes=1,1
  Signal Conversion : SignalConversion  OverrideOpt=off
  Subtract : Sum  Inputs=+-
  Switch : Switch  Criteria=u2 > Threshold  SaturateOnIntegerOverflow=off  InputSameDT=off
  Switch5 : Switch  Criteria=u2 > Threshold  Threshold=0.5  SaturateOnIntegerOverflow=off  InputSameDT=off
  TD : Subsystem
  Transpose1 : Math  Operator=transpose  SignedPower=on
  norm : Subsystem
  setpoint_next : Outport
  wires:
  Switch5/1 -> Signal Conversion/1
  Signal Conversion/1 -> TD/1(D)
  Constant11/1 -> TD/2(r)
  pos1/1 -> TD/3(r1), Subtract/1
  Transpose1/1 -> Subtract/2, Switch5/3
  TD/1(setpoint_next) -> setpoint_next/1
  FLAG/1 -> Switch5/2
  xyz_cmd/1 -> Switch5/1
  Constant5/1 -> Selector1/1
  Chart/1(flag_setpoint) -> Switch/2
  Subtract/1 -> norm/1(u)
  Add2/1 -> Saturation/1
  Switch/1 -> Add/1
  Constant2/1 -> Switch/3
  Memory/1 -> Add2/1, Add/2
  Constant1/1 -> Switch/1
  Constant4/1 -> Relational Operator2/2
  Saturation/1 -> Selector1/2
  Add/1 -> Memory/1
  Constant3/1 -> Add2/2
  Selector1/1 -> Transpose1/1
  norm/1(y) -> Relational Operator2/1
  Relational Operator2/1 -> Chart/1(dist)

== system THSDemo/NavigationModel/ Navigation Control （X,Y,Z）/SETPOINT_z1/takeoff1 ==
  posxy : Inport
  h : Inport  Port=2
  Enable : EnablePort
  Abs : Abs  SaturateOnIntegerOverflow=off
  Add : Sum  Inputs=+-
  Compare To Constant1 : simulink/Logic and Bit Operations/Compare To Constant  relop=<=  const=0.3  OutDataTypeStr=boolean
  Constant : Constant  Value=takeoff_h
  Constant5 : Constant  Value=setpoint1
  Memory : Memory
  Memory3 : Memory
  Mux : Mux  Inputs=2
  Mux1 : Mux  Inputs=2
  Switch : Switch  Criteria=u2 > Threshold  Threshold=0.5  SaturateOnIntegerOverflow=off  InputSameDT=off
  Switch1 : Switch  Criteria=u2 > Threshold  Threshold=0.5  SaturateOnIntegerOverflow=off  InputSameDT=off
  setpoint_next : Outport
  wires:
  Memory3/1 -> Switch1/2
  Compare To Constant1/1 -> Memory3/1, Switch/2
  Switch1/1 -> Compare To Constant1/1, Memory/1
  Memory/1 -> Switch1/1
  Mux1/1 -> Switch/3
  Mux/1 -> Switch/1
  Abs/1 -> Switch1/3
  Add/1 -> Abs/1
  h/1 -> Add/2
  posxy/1 -> Mux1/1
  Constant/1 -> Mux/2, Mux1/2, Add/1
  Constant5/1 -> Mux/1
  Switch/1 -> setpoint_next/1

== system THSDemo/NavigationModel/ Navigation Control （X,Y,Z）/SETPOINT_z1/takeoff2 ==
  posxy : Inport
  h : Inport  Port=2
  Enable : EnablePort
  Abs : Abs  SaturateOnIntegerOverflow=off
  Add : Sum  Inputs=+-
  Compare To Constant1 : simulink/Logic and Bit Operations/Compare To Constant  relop=<=  const=0.3  OutDataTypeStr=boolean
  Constant : Constant  Value=takeoff_h
  Constant5 : Constant  Value=setpoint1
  Memory : Memory
  Memory3 : Memory
  Mux : Mux  Inputs=2
  Mux1 : Mux  Inputs=2
  Switch : Switch  Criteria=u2 > Threshold  Threshold=0.5  SaturateOnIntegerOverflow=off  InputSameDT=off
  Switch1 : Switch  Criteria=u2 > Threshold  Threshold=0.5  SaturateOnIntegerOverflow=off  InputSameDT=off
  setpoint_next : Outport
  flag : Outport  Port=2
  wires:
  Switch/1 -> setpoint_next/1
  Constant5/1 -> Mux/1
  Constant/1 -> Add/1, Mux1/2, Mux/2
  posxy/1 -> Mux1/1
  h/1 -> Add/2
  Add/1 -> Abs/1
  Abs/1 -> Switch1/3
  Mux/1 -> Switch/1
  Mux1/1 -> Switch/3
  Memory/1 -> Switch1/1
  Switch1/1 -> Memory/1, Compare To Constant1/1
  Compare To Constant1/1 -> Switch/2, flag/1, Memory3/1
  Memory3/1 -> Switch1/2

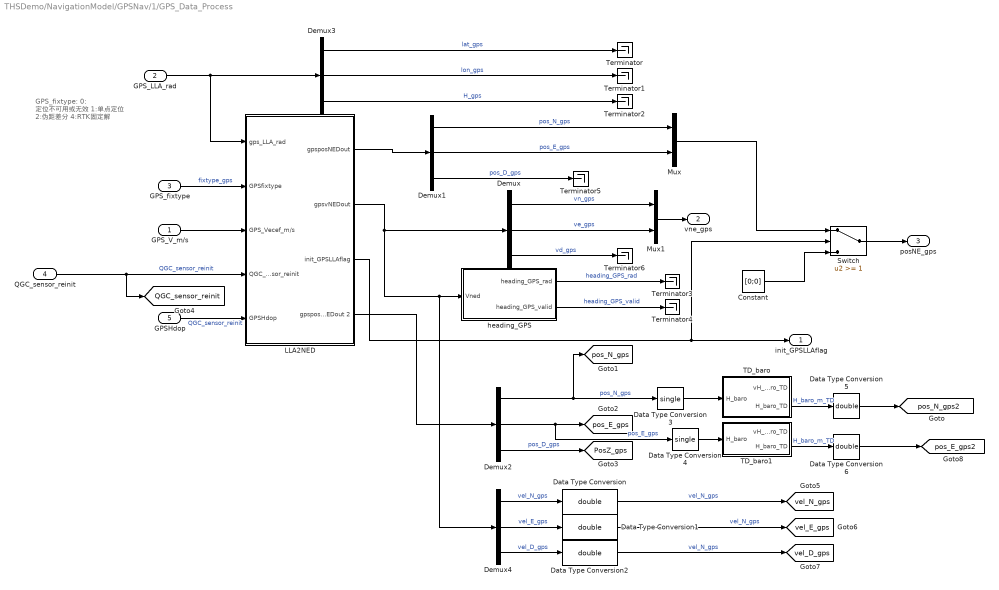
== system THSDemo/NavigationModel/GPSNav/1/GPS_Data_Process ==
  note: GPS_fixtype:
      | 0: 定位不可用或无效
      | 1:单点定位
      | 2:伪距差分
      | 4:RTK固定解
  GPS_V_m/s : Inport
  GPS_LLA_rad : Inport  Port=2
  GPS_fixtype : Inport  Port=3
  QGC_sensor_reinit : Inport  Port=4
  GPSHdop : Inport  Port=5
  Constant : Constant  Value=[0;0]
  Data Type Conversion{,1..2,5..6} (5 alike) : DataTypeConversion  OutDataTypeStr=double  SaturateOnIntegerOverflow=off  RndMeth=Floor
  Data Type Conversion3 : DataTypeConversion  OutDataTypeStr=single  SaturateOnIntegerOverflow=off  RndMeth=Floor
  Data Type Conversion4 : DataTypeConversion  OutDataTypeStr=single  SaturateOnIntegerOverflow=off  RndMeth=Floor
  Demux{,1..4} (5 alike) : Demux  Outputs=3
  LLA2NED : Subsystem
  Mux : Mux  Inputs=2
  Mux1 : Mux  Inputs=2
  Switch : Switch  Threshold=1  SaturateOnIntegerOverflow=off  InputSameDT=off
  TD_baro : Subsystem
  TD_baro1 : Subsystem
  Terminator{,1..6} (7 alike) : Terminator
  heading_GPS : Subsystem
  init_GPSLLAflag : Outport
  vne_gps : Outport  Port=2
  posNE_gps : Outport  Port=3
  tag scope: PosZ_gps=global, QGC_sensor_reinit=global, pos_E_gps2=global, pos_E_gps=global, pos_N_gps2=global, pos_N_gps=global, vel_D_gps=global, vel_E_gps=global, vel_N_gps=global
  wires:
  GPS_fixtype/1 -> LLA2NED/2(GPSfixtype)  "fixtype_gps"
  Demux3/3 -> Terminator2/1  "H_gps"
  Demux/3 -> Terminator6/1  "vd_gps"
  Demux/1 -> Mux1/1  "vn_gps"
  GPS_LLA_rad/1 -> Demux3/1, LLA2NED/1(gps_LLA_rad)
  Demux/2 -> Mux1/2  "ve_gps"
  Demux3/2 -> Terminator1/1  "lon_gps"
  Demux3/1 -> Terminator/1  "lat_gps"
  QGC_sensor_reinit/1 -> [QGC_sensor_reinit], LLA2NED/4(QGC_sensor_reinit)  "QGC_sensor_reinit"
  LLA2NED/1("gpsposNEDout ") -> Demux1/1
  Demux1/1 -> Mux/1  "pos_N_gps"
  Demux1/2 -> Mux/2  "pos_E_gps"
  Demux1/3 -> Terminator5/1  "pos_D_gps"
  GPS_V_m/s/1 -> LLA2NED/3(GPS_Vecef_m/s)
  LLA2NED/2(gpsvNEDout) -> Demux4/1, heading_GPS/1(Vned), Demux/1
  heading_GPS/1(heading_GPS_rad) -> Terminator3/1  "heading_GPS_rad"
  heading_GPS/2(heading_GPS_valid) -> Terminator4/1  "heading_GPS_valid"
  Mux/1 -> Switch/1
  Mux1/1 -> vne_gps/1
  GPSHdop/1 -> LLA2NED/5(GPSHdop)  "QGC_sensor_reinit"
  LLA2NED/3(init_GPSLLAflag) -> Switch/2, init_GPSLLAflag/1
  Constant/1 -> Switch/3
  Switch/1 -> posNE_gps/1
  Demux2/1 -> [pos_N_gps], Data Type Conversion3/1  "pos_N_gps"
  Demux2/3 -> [PosZ_gps]  "pos_D_gps"
  Demux2/2 -> Data Type Conversion4/1, [pos_E_gps]  "pos_E_gps"
  LLA2NED/4(gpsposNEDout 2) -> Demux2/1
  Demux4/2 -> Data Type Conversion1/1  "vel_E_gps"
  Demux4/3 -> Data Type Conversion2/1  "vel_D_gps"
  Demux4/1 -> Data Type Conversion/1  "vel_N_gps"
  Data Type Conversion/1 -> [vel_N_gps]  "vel_N_gps"
  Data Type Conversion1/1 -> [vel_E_gps]  "vel_N_gps"
  Data Type Conversion2/1 -> [vel_D_gps]  "vel_N_gps"
  TD_baro/2(H_baro_TD) -> Data Type Conversion5/1  "H_baro_m_TD"
  TD_baro1/2(H_baro_TD) -> Data Type Conversion6/1  "H_baro_m_TD"
  Data Type Conversion3/1 -> TD_baro/1(H_baro)
  Data Type Conversion4/1 -> TD_baro1/1(H_baro)
  Data Type Conversion5/1 -> [pos_N_gps2]
  Data Type Conversion6/1 -> [pos_E_gps2]

== system THSDemo/NavigationModel/GPSNav/1/Translation_estimate ==
  Cbn : Inport
  accl_ned_m/s2 : Inport  Port=2
  vne_gps : Inport  Port=3
  posNE_gps1 : Inport  Port=4
  GPSstate : Inport  Port=5
  GPSHdop : Inport  Port=6
  QGC_init : Inport  Port=7
  Enable : EnablePort
  Subsystem : Subsystem
  Subsystem2 : Subsystem
  V_Horizontal_estimation1 : Subsystem  Commented=on
  translate to N : Subsystem
  vxy_estimout : Outport
  Pxy_estimout : Outport  Port=2
  wires:
  Cbn/1 -> translate to N/1(Cbn)
  accl_ned_m/s2/1 -> translate to N/2(accl_ned)
  QGC_init/1 -> Subsystem/4(QGC_init), Subsystem2/3(QGC_init)
  posNE_gps1/1 -> Subsystem/2(pxy_GPS)
  GPSHdop/1 -> Subsystem2/4(DOP), Subsystem/5(DOP)
  Subsystem/1(pxy_est) -> Pxy_estimout/1
  Subsystem2/1(vxy_est) -> vxy_estimout/1, Subsystem/1(vxy)
  translate to N/1(accel_Horizontal_predict) -> Subsystem2/1(axy)
  vne_gps/1 -> Subsystem2/2(vxy_GPS)
  Subsystem2/2(GPSv_enable) -> Subsystem/3(GPSv_enable)

== system THSDemo/NavigationModel/ Navigation Control （X,Y,Z）/SETPOINT_z1/return_mode1/TD ==
  D : Inport
  r : Inport  Port=2
  r1 : Inport  Port=3
  Constant1 : Constant  Value=0.01
  Discrete-Time Integrator1 : DiscreteIntegrator  InitialConditionSource=external  SampleTime=-1  ICPrevOutput=DiscIntNeverNeededParam  ICPrevScaledInput=DiscIntNeverNeededParam
  Discrete-Time Integrator3 : DiscreteIntegrator  SampleTime=-1  ICPrevOutput=DiscIntNeverNeededParam  ICPrevScaledInput=DiscIntNeverNeededParam
  Fhan : Subsystem
  Sum24 : Sum  Inputs=|-+
  x1 : Scope
  x2 : Scope
  setpoint_next : Outport
  wires:
  Fhan/1(fh) -> Discrete-Time Integrator3/1
  Constant1/1 -> Fhan/4(h)
  Discrete-Time Integrator1/1 -> setpoint_next/1, Sum24/2, x1/1  "x1"
  D/1 -> Sum24/1
  Sum24/1 -> Fhan/1(x1)
  Discrete-Time Integrator3/1 -> x2/1, Discrete-Time Integrator1/1, Fhan/2(x2)  "x2"
  r/1 -> Fhan/3(r)
  r1/1 -> Discrete-Time Integrator1/2

== system THSDemo/NavigationModel/ Navigation Control （X,Y,Z）/SETPOINT_z1/return_mode1/norm ==
  u : Inport
  Product : Product
  Sqrt : Sqrt
  Sum of Elements : Sum  Inputs=+
  y : Outport
  wires:
  Sum of Elements/1 -> Sqrt/1
  Product/1 -> Sum of Elements/1
  u/1 -> Product/2, Product/1
  Sqrt/1 -> y/1

== system THSDemo/NavigationModel/ Navigation Control （X,Y,Z）/SETPOINT_z1/return_mode2/TD ==
  D : Inport
  r : Inport  Port=2
  r1 : Inport  Port=3
  Constant1 : Constant  Value=0.01
  Discrete-Time Integrator1 : DiscreteIntegrator  InitialConditionSource=external  SampleTime=-1  ICPrevOutput=DiscIntNeverNeededParam  ICPrevScaledInput=DiscIntNeverNeededParam
  Discrete-Time Integrator3 : DiscreteIntegrator  SampleTime=-1  ICPrevOutput=DiscIntNeverNeededParam  ICPrevScaledInput=DiscIntNeverNeededParam
  Fhan : Subsystem
  Sum24 : Sum  Inputs=|-+
  x1 : Scope
  x2 : Scope
  setpoint_next : Outport
  wires:
  r1/1 -> Discrete-Time Integrator1/2
  r/1 -> Fhan/3(r)
  Discrete-Time Integrator3/1 -> Fhan/2(x2), Discrete-Time Integrator1/1, x2/1  "x2"
  Sum24/1 -> Fhan/1(x1)
  D/1 -> Sum24/1
  Discrete-Time Integrator1/1 -> x1/1, Sum24/2, setpoint_next/1  "x1"
  Constant1/1 -> Fhan/4(h)
  Fhan/1(fh) -> Discrete-Time Integrator3/1

== system THSDemo/NavigationModel/ Navigation Control （X,Y,Z）/SETPOINT_z1/return_mode2/norm ==
  u : Inport
  Product : Product
  Sqrt : Sqrt
  Sum of Elements : Sum  Inputs=+
  y : Outport
  wires:
  Sqrt/1 -> y/1
  u/1 -> Product/1, Product/2
  Product/1 -> Sum of Elements/1
  Sum of Elements/1 -> Sqrt/1

== system THSDemo/NavigationModel/ Navigation Control （X,Y,Z）/SETPOINT_z1/setpoints1/TD ==
  D : Inport
  r : Inport  Port=2
  r1 : Inport  Port=3
  Constant1 : Constant  Value=0.01
  Discrete-Time Integrator1 : DiscreteIntegrator  InitialConditionSource=external  SampleTime=-1  ICPrevOutput=DiscIntNeverNeededParam  ICPrevScaledInput=DiscIntNeverNeededParam
  Discrete-Time Integrator3 : DiscreteIntegrator  SampleTime=-1  ICPrevOutput=DiscIntNeverNeededParam  ICPrevScaledInput=DiscIntNeverNeededParam
  Fhan : Subsystem
  Sum24 : Sum  Inputs=|-+
  x1 : Scope
  x2 : Scope
  setpoint_next : Outport
  wires:
  Fhan/1(fh) -> Discrete-Time Integrator3/1
  Constant1/1 -> Fhan/4(h)
  Discrete-Time Integrator1/1 -> setpoint_next/1, Sum24/2, x1/1  "x1"
  D/1 -> Sum24/1
  Sum24/1 -> Fhan/1(x1)
  Discrete-Time Integrator3/1 -> x2/1, Discrete-Time Integrator1/1, Fhan/2(x2)  "x2"
  r/1 -> Fhan/3(r)
  r1/1 -> Discrete-Time Integrator1/2

== system THSDemo/NavigationModel/ Navigation Control （X,Y,Z）/SETPOINT_z1/setpoints1/norm ==
  u : Inport
  Product : Product
  Sqrt : Sqrt
  Sum of Elements : Sum  Inputs=+
  y : Outport
  wires:
  Sum of Elements/1 -> Sqrt/1
  Product/1 -> Sum of Elements/1
  u/1 -> Product/2, Product/1
  Sqrt/1 -> y/1

== system THSDemo/NavigationModel/ Navigation Control （X,Y,Z）/SETPOINT_z1/setpoints2/TD ==
  D : Inport
  r : Inport  Port=2
  r1 : Inport  Port=3
  Constant1 : Constant  Value=0.01
  Discrete-Time Integrator1 : DiscreteIntegrator  InitialConditionSource=external  SampleTime=-1  ICPrevOutput=DiscIntNeverNeededParam  ICPrevScaledInput=DiscIntNeverNeededParam
  Discrete-Time Integrator3 : DiscreteIntegrator  SampleTime=-1  ICPrevOutput=DiscIntNeverNeededParam  ICPrevScaledInput=DiscIntNeverNeededParam
  Fhan : Subsystem
  Sum24 : Sum  Inputs=|-+
  x1 : Scope
  x2 : Scope
  setpoint_next : Outport
  wires:
  r1/1 -> Discrete-Time Integrator1/2
  r/1 -> Fhan/3(r)
  Discrete-Time Integrator3/1 -> Fhan/2(x2), Discrete-Time Integrator1/1, x2/1  "x2"
  Sum24/1 -> Fhan/1(x1)
  D/1 -> Sum24/1
  Discrete-Time Integrator1/1 -> x1/1, Sum24/2, setpoint_next/1  "x1"
  Constant1/1 -> Fhan/4(h)
  Fhan/1(fh) -> Discrete-Time Integrator3/1

== system THSDemo/NavigationModel/ Navigation Control （X,Y,Z）/SETPOINT_z1/setpoints2/norm ==
  u : Inport
  Product : Product
  Sqrt : Sqrt
  Sum of Elements : Sum  Inputs=+
  y : Outport
  wires:
  Sqrt/1 -> y/1
  u/1 -> Product/1, Product/2
  Product/1 -> Sum of Elements/1
  Sum of Elements/1 -> Sqrt/1
